simulink model "scheme"  (R2026b)
settings: Solver=ode45  StopTime=25  MaxStep=0.001  RelTol=1e-9  AbsTol=1e-11
settings Model: Creator=Asus  LastModifiedBy=Asus
settings DataIOCC: OutputOption=SpecifiedOutputTimes  OutputTimes=0:0.001:25  SaveOutput=off

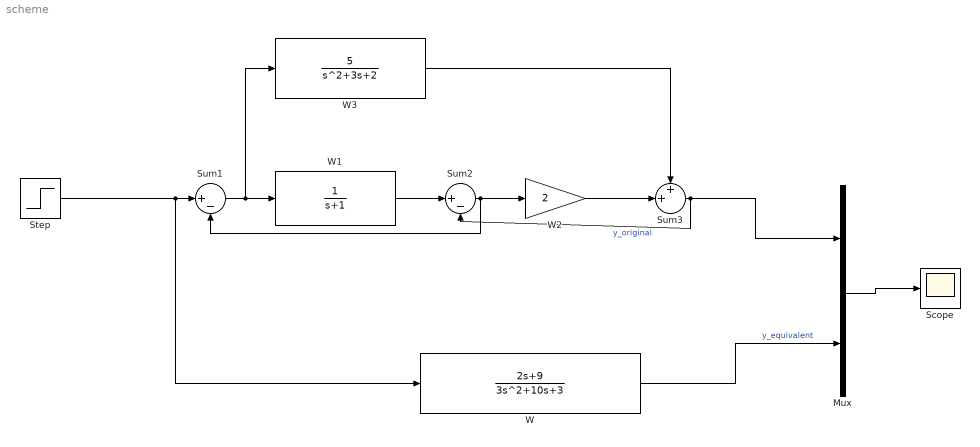
== system scheme ==
  Mux : Mux  Inputs=2
  Scope : Scope
      settings: TimeSpan=25  ActiveDisplayYMinimum=-0.374906105673273  ActiveDisplayYMaximum=3.3741549510594573  YLabel=y(t)  DataLoggingVariableName=scopeData
  Step : Step  Time=0  SampleTime=0
  Sum1 : Sum  Inputs=|+-
  Sum2 : Sum  Inputs=|+-
  Sum3 : Sum  Inputs=++|
  W : TransferFcn  Numerator=[2 9]  Denominator=[3 10 3]
  W1 : TransferFcn  Numerator=1  Denominator=[1 1]
  W2 : Gain  Gain=2
  W3 : TransferFcn  Numerator=5  Denominator=[1 3 2]
  wires:
  Sum1/1 -> W1/1, W3/1
  W1/1 -> Sum2/1
  Sum2/1 -> W2/1, Sum1/2
  W2/1 -> Sum3/2
  W3/1 -> Sum3/1
  Sum3/1 -> Mux/1, Sum2/2  "y_original"
  W/1 -> Mux/2  "y_equivalent"
  Mux/1 -> Scope/1
  Step/1 -> Sum1/1, W/1
